simulink library "traj_lib"  (R2018b)
settings: Solver=VariableStepAuto  StartTime=0.0  StopTime=10.0  RelTol=1e-3
undefined symbols (not defined in the file or in its folder): traj_empty_struct, traj_params
libraries: $bdroot x1, simulink x1
settings Model: Creator=fabian  LastModifiedBy=yannic

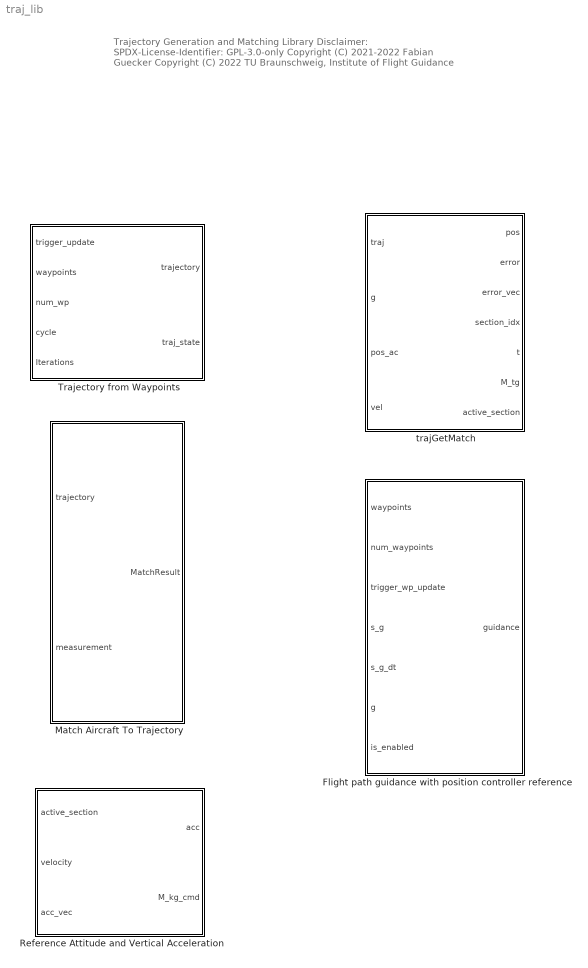
== system traj_lib ==
  note: Trajectory Generation and Matching Library
      |
      | Disclaimer:
      | SPDX-License-Identifier: GPL-3.0-only
      |
      | Copyright (C) 2021-2022 Fabian Guecker
      | Copyright (C) 2022 TU Braunschweig, Institute of Flight Guidance
  Flight path guidance with position controller reference : Subsystem  mask{traj_params=traj_params, T_inner_loop=0.1, mask_expr_handling_config=default}
      mask prompts: traj_params "Guided flight mode parameters struct"; T_inner_loop "Inner loop time constant seen by position controller, in s"
      mask init:
      | maskExprHandling(gcbh, mask_expr_handling_config);
      mask TypeOptions mask_expr_handling_config: default | passthrough (tunable)
      mask DialogControl DescGroupVar Prompt: Position controller reference from waypoints
      mask DialogControl DescTextVar Prompt: Waypoints are connected by splines. The shortest distance to the desired flight path is computed. Then the corresponding desired position, velocity and acceleration are computed based on the desired flight-path velocity.
      mask DialogControl CodeGenerationSettings Prompt: Code Generation Settings
      mask DialogControl maskExprHandlingText Prompt: Mask expression handling
      mask DialogControl maskExprHandlingReadme Prompt: README
      mask DialogControl maskExprHandlingReadme Tooltip: https://github.com/iff-gsc/m-Utils/tree/main/simulink/mask_expression_handling/README.md
      mask DialogControl maskExprHandlingReadme Callback: web('https://github.com/iff-gsc/m-Utils/tree/main/simulink/mask_expression_handling/README.md','-browser')
  Match Aircraft To Trajectory : Subsystem
      mask DialogControl DescGroupVar Prompt: Match Aircraft to Trajectory
  Reference Attitude and Vertical Acceleration : Subsystem  mask{G0=9.81}
      mask prompts: G0 "earth acceleration [m/s^2]"
  Trajectory from Waypoints : Subsystem  mask{traj_parameter=traj_params}
      mask prompts: traj_parameter "Trajectory parameters struct, see trajLoadParams"
      mask init:
      | [traj_empty_struct] = trajInit(traj_parameter.wpmax, traj_parameter.degree);
      | struct2slbus( traj_empty_struct, 'trajectoryStruct' );
      mask DialogControl DescGroupVar Prompt: Trajectory from Waypoints
  trajGetMatch : MATLAB Function  TreatAsAtomicUnit=on

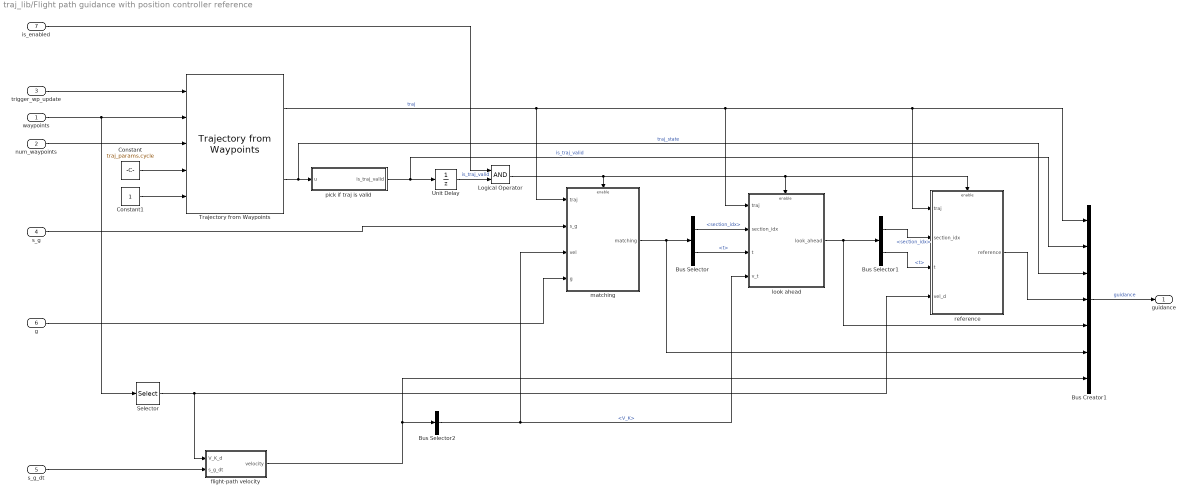
== system traj_lib/Flight path guidance with position controller reference ==
  waypoints : Inport
  num_waypoints : Inport  Port=2
  trigger_wp_update : Inport  Port=3
  s_g : Inport  Port=4
  s_g_dt : Inport  Port=5
  g : Inport  Port=6
  is_enabled : Inport  Port=7
  Bus Creator1 : BusCreator  Inputs=7
  Bus Selector : BusSelector  OutputSignals=section_idx,t
  Bus Selector1 : BusSelector  OutputSignals=section_idx,t
  Bus Selector2 : BusSelector  OutputSignals=V_K
  Constant : Constant  Value=traj_params.cycle
  Constant1 : Constant
  Logical Operator : Logic  AllPortsSameDT=off  OutDataTypeStr=boolean
  Selector : Selector  NumberOfDimensions=2  InputPortWidth=3  IndexOptions=Index vector (dialog),Index vector (dialog)  Indices=4,1  OutputSizes=1,1
  Trajectory from Waypoints : $bdroot/Trajectory from Waypoints  traj_parameter=traj_params
  Unit Delay : UnitDelay  SampleTime=-1
  flight-path velocity : Subsystem
  look ahead : Subsystem
  matching : Subsystem
  pick if traj is valid : MATLAB Function  TreatAsAtomicUnit=on
  reference : Subsystem
  guidance : Outport
  wires:
  waypoints/1 -> Selector/1, Trajectory from Waypoints/2
  g/1 -> matching/4(g)
  Constant/1 -> Trajectory from Waypoints/4
  Trajectory from Waypoints/1 -> matching/1(traj), look ahead/1(traj), reference/1(traj), Bus Creator1/1  "traj"
  s_g/1 -> matching/2(s_g)
  matching/1(matching) -> Bus Creator1/6, Bus Selector/1
  Selector/1 -> flight-path velocity/1(V_K_d), reference/4(vel_d)
  look ahead/1(look_ahead) -> Bus Creator1/5, Bus Selector1/1
  reference/1(reference) -> Bus Creator1/4
  Bus Selector/1 -> look ahead/2(section_idx)  "<section_idx>"
  Bus Selector/2 -> look ahead/3(t)  "<t>"
  Bus Selector1/1 -> reference/2(section_idx)  "<section_idx>"
  Bus Selector1/2 -> reference/3(t)  "<t>"
  Bus Creator1/1 -> guidance/1  "guidance"
  s_g_dt/1 -> flight-path velocity/2(s_g_dt)
  flight-path velocity/1(velocity) -> Bus Creator1/7, Bus Selector2/1
  Bus Selector2/1 -> look ahead/4(v_t), matching/3(vel)  "<V_K>"
  Constant1/1 -> Trajectory from Waypoints/5
  num_waypoints/1 -> Trajectory from Waypoints/3
  Trajectory from Waypoints/2 -> Bus Creator1/3, pick if traj is valid/1(u)  "traj_state"
  pick if traj is valid/1(is_traj_valid) -> Unit Delay/1, Bus Creator1/2  "is_traj_valid"
  Logical Operator/1 -> matching/Enable, look ahead/Enable, reference/Enable
  trigger_wp_update/1 -> Trajectory from Waypoints/1
  is_enabled/1 -> Logical Operator/1
  Unit Delay/1 -> Logical Operator/2  "is_traj_valid"

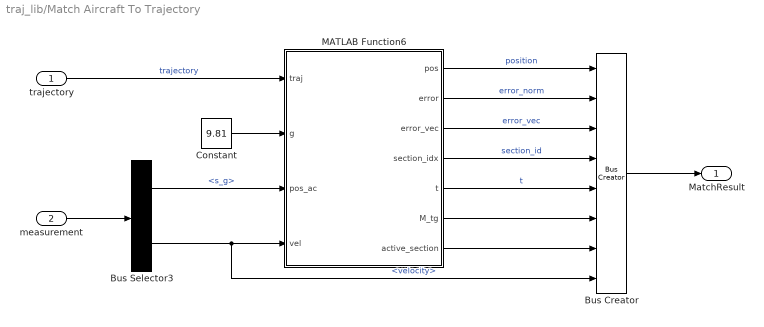
== system traj_lib/Match Aircraft To Trajectory ==
  trajectory : Inport
  measurement : Inport  Port=2
  Bus Creator : BusCreator  Inputs=8
  Bus Selector3 : BusSelector  OutputSignals=EKF.s_g,EKF.velocity
  Constant : Constant  Value=9.81
  MATLAB Function6 : MATLAB Function  TreatAsAtomicUnit=on
  MatchResult : Outport
  wires:
  Bus Selector3/1 -> MATLAB Function6/3(pos_ac)  "<s_g>"
  trajectory/1 -> MATLAB Function6/1(traj)  "trajectory"
  measurement/1 -> Bus Selector3/1
  Bus Creator/1 -> MatchResult/1
  Bus Selector3/2 -> Bus Creator/8, MATLAB Function6/4(vel)  "<velocity>"
  Constant/1 -> MATLAB Function6/2(g)
  MATLAB Function6/1(pos) -> Bus Creator/1  "position"
  MATLAB Function6/2(error) -> Bus Creator/2  "error_norm"
  MATLAB Function6/3(error_vec) -> Bus Creator/3  "error_vec"
  MATLAB Function6/4(section_idx) -> Bus Creator/4  "section_id"
  MATLAB Function6/5(t) -> Bus Creator/5  "t"
  MATLAB Function6/6(M_tg) -> Bus Creator/6
  MATLAB Function6/7(active_section) -> Bus Creator/7

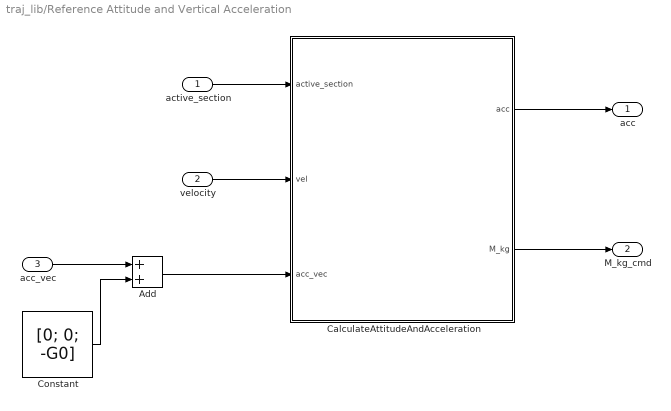
== system traj_lib/Reference Attitude and Vertical Acceleration ==
  active_section : Inport
  velocity : Inport  Port=2
  acc_vec : Inport  Port=3
  Add : Sum
  CalculateAttitudeAndAcceleration : MATLAB Function  TreatAsAtomicUnit=on
  Constant : Constant  Value=[0; 0; -G0]  VectorParams1D=off
  acc : Outport
  M_kg_cmd : Outport  Port=2
  wires:
  active_section/1 -> CalculateAttitudeAndAcceleration/1(active_section)
  velocity/1 -> CalculateAttitudeAndAcceleration/2(vel)
  CalculateAttitudeAndAcceleration/2(M_kg) -> M_kg_cmd/1
  Constant/1 -> Add/2
  CalculateAttitudeAndAcceleration/1(acc) -> acc/1
  acc_vec/1 -> Add/1
  Add/1 -> CalculateAttitudeAndAcceleration/3(acc_vec)

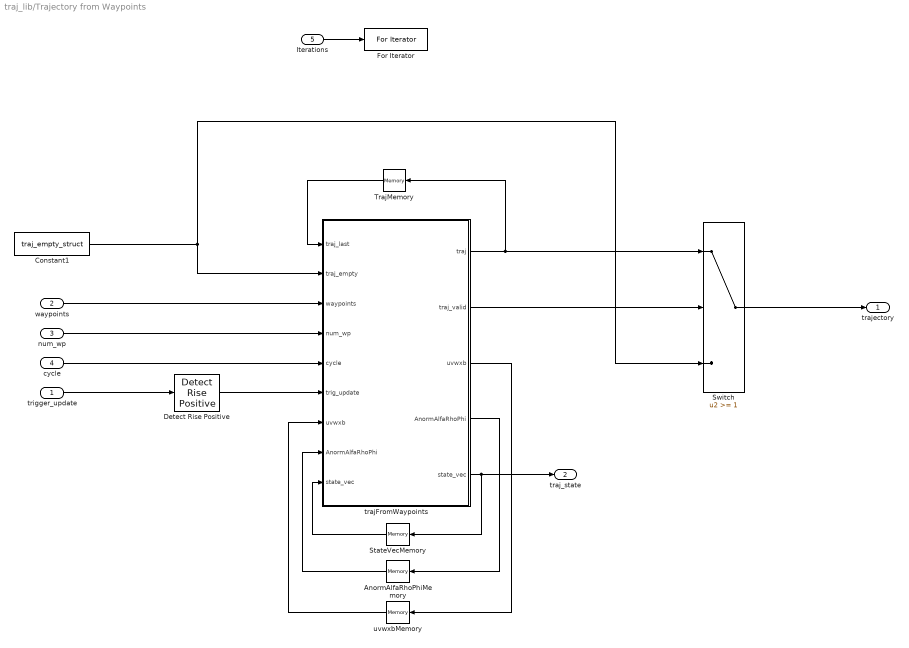
== system traj_lib/Trajectory from Waypoints ==
  trigger_update : Inport
  waypoints : Inport  Port=2
  num_wp : Inport  Port=3
  cycle : Inport  Port=4
  Iterations : Inport  Port=5  OutMin=[1]  OutMax=[100]  PortDimensions=1
  AnormAlfaRhoPhiMemory : Memory  InitialCondition=zeros(4,1)  InheritSampleTime=on
  Constant1 : Constant  Value=traj_empty_struct  OutDataTypeStr=Bus: trajectoryStructBus
  Detect Rise Positive : simulink/Logic and Bit Operations/Detect Rise Positive  vinit=0  OutDataTypeStr=boolean
  For Iterator : ForIterator  IterationSource=external  IterationLimit=100  ShowIterationPort=off
  "StateVecMemory " : Memory  InitialCondition=zeros(6,1)  InheritSampleTime=on
  Switch : Switch  Threshold=1
  TrajMemory : Memory  InitialCondition=traj_empty_struct  InheritSampleTime=on
  trajFromWaypoints : MATLAB Function  TreatAsAtomicUnit=on
  uvwxbMemory : Memory  InitialCondition=zeros(traj_parameter.wpmax*(traj_parameter.degree+1),5)  InheritSampleTime=on
  trajectory : Outport
  traj_state : Outport  Port=2
  wires:
  AnormAlfaRhoPhiMemory/1 -> trajFromWaypoints/8("AnormAlfaRhoPhi ")
  Switch/1 -> trajectory/1
  Iterations/1 -> For Iterator/1
  num_wp/1 -> trajFromWaypoints/4(num_wp)
  waypoints/1 -> trajFromWaypoints/3(waypoints)
  TrajMemory/1 -> trajFromWaypoints/1(traj_last)
  Detect Rise Positive/1 -> trajFromWaypoints/6(trig_update)
  cycle/1 -> trajFromWaypoints/5(cycle)
  Constant1/1 -> trajFromWaypoints/2(traj_empty), Switch/3
  uvwxbMemory/1 -> trajFromWaypoints/7("uvwxb ")
  "StateVecMemory "/1 -> trajFromWaypoints/9("state_vec ")
  trajFromWaypoints/5(state_vec) -> traj_state/1, "StateVecMemory "/1
  trajFromWaypoints/2(traj_valid) -> Switch/2
  trigger_update/1 -> Detect Rise Positive/1
  trajFromWaypoints/1(traj) -> TrajMemory/1, Switch/1
  trajFromWaypoints/4(AnormAlfaRhoPhi) -> AnormAlfaRhoPhiMemory/1
  trajFromWaypoints/3(uvwxb) -> uvwxbMemory/1

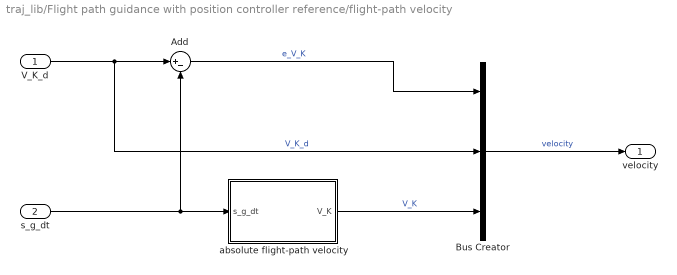
== system traj_lib/Flight path guidance with position controller reference/flight-path velocity ==
  V_K_d : Inport
  s_g_dt : Inport  Port=2
  Add : Sum  Inputs=|+-
  Bus Creator : BusCreator  Inputs=3
  absolute flight-path velocity : Subsystem
  velocity : Outport
  wires:
  s_g_dt/1 -> absolute flight-path velocity/1(s_g_dt), Add/2
  absolute flight-path velocity/1(V_K) -> Bus Creator/3  "V_K"
  V_K_d/1 -> Bus Creator/2, Add/1  "V_K_d"
  Bus Creator/1 -> velocity/1  "velocity"
  Add/1 -> Bus Creator/1  "e_V_K"

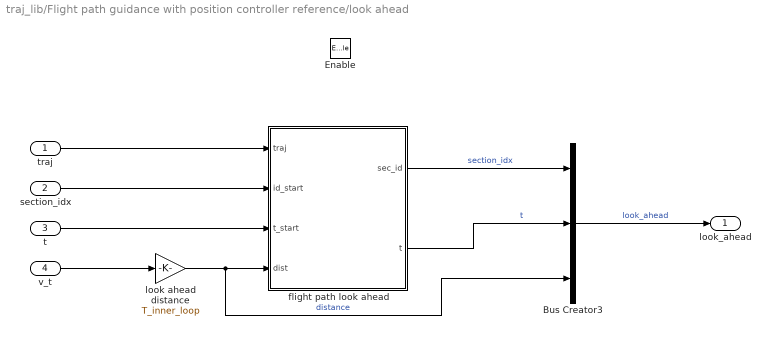
== system traj_lib/Flight path guidance with position controller reference/look ahead ==
  traj : Inport
  section_idx : Inport  Port=2
  t : Inport  Port=3
  v_t : Inport  Port=4
  Enable : EnablePort
  Bus Creator3 : BusCreator  Inputs=3
  flight path look ahead : MATLAB Function  TreatAsAtomicUnit=on
  look ahead distance : Gain  Gain=T_inner_loop
  look_ahead : Outport
  wires:
  v_t/1 -> look ahead distance/1
  flight path look ahead/2(t) -> Bus Creator3/2  "t"
  Bus Creator3/1 -> look_ahead/1  "look_ahead"
  section_idx/1 -> flight path look ahead/2(id_start)
  traj/1 -> flight path look ahead/1(traj)
  flight path look ahead/1(sec_id) -> Bus Creator3/1  "section_idx"
  t/1 -> flight path look ahead/3(t_start)
  look ahead distance/1 -> Bus Creator3/3, flight path look ahead/4(dist)  "distance"

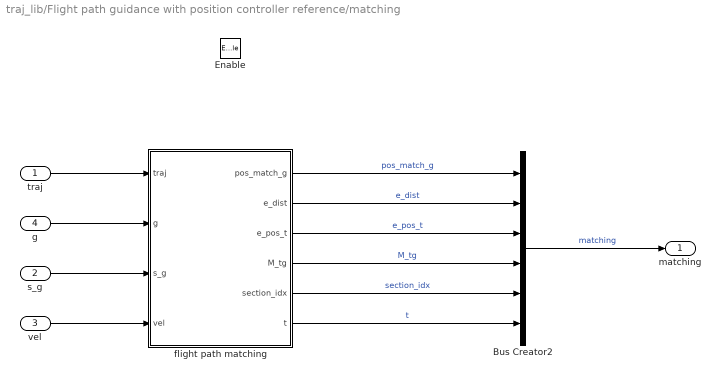
== system traj_lib/Flight path guidance with position controller reference/matching ==
  traj : Inport
  s_g : Inport  Port=2
  vel : Inport  Port=3
  g : Inport  Port=4
  Enable : EnablePort
  Bus Creator2 : BusCreator  Inputs=6
  flight path matching : MATLAB Function  TreatAsAtomicUnit=on
  matching : Outport
  wires:
  flight path matching/5(section_idx) -> Bus Creator2/5  "section_idx"
  traj/1 -> flight path matching/1(traj)
  flight path matching/3(e_pos_t) -> Bus Creator2/3  "e_pos_t"
  flight path matching/6(t) -> Bus Creator2/6  "t"
  g/1 -> flight path matching/2(g)
  flight path matching/1(pos_match_g) -> Bus Creator2/1  "pos_match_g"
  vel/1 -> flight path matching/4(vel)
  flight path matching/2(e_dist) -> Bus Creator2/2  "e_dist"
  s_g/1 -> flight path matching/3(s_g)
  Bus Creator2/1 -> matching/1  "matching"
  flight path matching/4(M_tg) -> Bus Creator2/4  "M_tg"

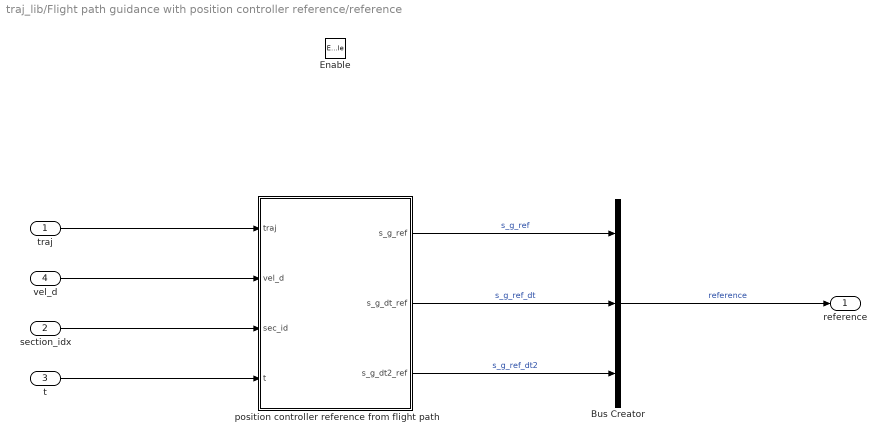
== system traj_lib/Flight path guidance with position controller reference/reference ==
  traj : Inport
  section_idx : Inport  Port=2
  t : Inport  Port=3
  vel_d : Inport  Port=4
  Enable : EnablePort
  Bus Creator : BusCreator  Inputs=3
  position controller reference from flight path : MATLAB Function  TreatAsAtomicUnit=on
  reference : Outport
  wires:
  position controller reference from flight path/1(s_g_ref) -> Bus Creator/1  "s_g_ref"
  vel_d/1 -> position controller reference from flight path/2(vel_d)
  position controller reference from flight path/2(s_g_dt_ref) -> Bus Creator/2  "s_g_ref_dt"
  t/1 -> position controller reference from flight path/4(t)
  position controller reference from flight path/3(s_g_dt2_ref) -> Bus Creator/3  "s_g_ref_dt2"
  traj/1 -> position controller reference from flight path/1(traj)
  Bus Creator/1 -> reference/1  "reference"
  section_idx/1 -> position controller reference from flight path/3(sec_id)

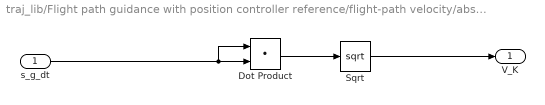
== system traj_lib/Flight path guidance with position controller reference/flight-path velocity/absolute flight-path velocity ==
  s_g_dt : Inport
  Dot Product : DotProduct  InputSameDT=on  OutDataTypeStr=Inherit: Inherit via internal rule
  Sqrt : Sqrt  SaturateOnIntegerOverflow=on
  V_K : Outport
  wires:
  Dot Product/1 -> Sqrt/1
  Sqrt/1 -> V_K/1
  s_g_dt/1 -> Dot Product/1, Dot Product/2

== matlab function traj_lib/trajGetMatch ==
  data: pos output; error output; error_vec output; traj input; g input; pos_ac input; section_idx output; t output; M_tg output; vel input; active_section output Bus: sections
function [pos, error, error_vec, section_idx, t, M_tg, active_section]  = GetMatch(traj, g, pos_ac, vel)

    section_idx = ones(1,superiorfloat(pos_ac));

    [section_idx, error, t] = trajGetMatchEnhanced(traj, pos_ac, section_idx);
    
    active_section   = trajGetSection(traj, section_idx);
    active_section.t = t;
    
    pos = trajSectionGetPos(active_section);
         
    error_vec = (pos - pos_ac);  

    [T, B, N, ~, ~] = trajSectionGetFrenetSerretWithGravity(active_section, vel, g);

    M_tg = [T, B, -N];

end

== matlab function traj_lib/Match Aircraft To Trajectory/MATLAB Function6 ==
  data: pos output; error output; error_vec output; traj input; g input; pos_ac input; section_idx output; t output; M_tg output; vel input; active_section output Bus: sections
function [pos, error, error_vec, section_idx, t, M_tg, active_section]  = GetMatch(traj, g, pos_ac, vel)

    section_idx = 1;

    [section_idx, error, t] = trajGetMatch(traj, pos_ac, section_idx);
    
    active_section   = trajGetSection(traj, section_idx);
    active_section.t = t;
    
    pos = trajSectionGetPos(active_section);
         
    error_vec = (pos - pos_ac);  

    [T, B, N, ~, ~] = trajSectionGetFrenetSerretWithGravity(active_section, vel, g);

    M_tg = [T, B, -N];

end

== matlab function traj_lib/Flight path guidance with position controller reference/pick if traj is valid ==
  data: u input; is_traj_valid output
function is_traj_valid = fcn(u)
is_traj_valid = u(5);
end

== matlab function traj_lib/Flight path guidance with position controller reference/matching/flight path matching ==
  data: pos_match_g output; e_dist output; e_pos_t output; M_tg output; traj input size=1; section_idx output size=1; g input size=1; s_g input size=3; vel input size=1; t output size=1
function [pos_match_g, e_dist, e_pos_t, M_tg, section_idx, t]  = fcn(traj, g, s_g, vel)

    [section_idx, e_dist, t] = trajGetMatchEnhanced(traj, s_g);
    
    traj_section   = trajGetSection(traj, section_idx);
    
    pos_match_g = trajSectionGetPos(traj_section,t);
    
    [T, B, N, ~, ~] = trajSectionGetFrenetSerretWithGravity(traj_section, vel, g, t);
    M_tg = [T, B, -N]';
         
    e_pos_t = M_tg * (pos_match_g - s_g);  
    
end

== matlab function traj_lib/Flight path guidance with position controller reference/reference/position controller reference from flight path ==
  data: traj input; vel_d input; s_g_ref output size=3; s_g_dt_ref output; sec_id input; t input; s_g_dt2_ref output
function [s_g_ref,s_g_dt_ref,s_g_dt2_ref] = fcn(traj, vel_d, sec_id, t)
traj_section = trajGetSection(traj,sec_id);
s_g_ref = trajSectionGetPos(traj_section,t);
s_g_dt_ref = trajSectionGetVel(traj_section,vel_d,t);
s_g_dt2_ref = trajSectionGetAcc(traj_section,vel_d,0, t);
end

== matlab function traj_lib/Flight path guidance with position controller reference/look ahead/flight path look ahead ==
  data: traj input; sec_id output size=1; id_start input size=1; t_start input; dist input; t output size=1
function [sec_id,t] = trajSweepAlong(traj,id_start,t_start,dist)
[sec_id, t] = trajSweepAlong(traj,id_start,t_start,dist);
end

== matlab function traj_lib/Reference Attitude and Vertical Acceleration/CalculateAttitudeAndAcceleration ==
  data: active_section input; vel input; acc output; M_kg output; acc_vec input
function [acc, M_kg] = CalculateAttitudeAndAcceleration(active_section, vel, acc_vec)

[T, B, N, kappa, ~] = trajSectionGetFrenetSerretWithAcceleration(active_section, vel, acc_vec);

% Calculate path acceleration
acc = (kappa * N) * vel^2;

M_kg = [T, B, -N];

end

== matlab function traj_lib/Trajectory from Waypoints/trajFromWaypoints ==
  settings: updateMethod=DISCRETE
  data: traj_last input; traj_empty input; waypoints input; num_wp input; cycle input; trig_update input; uvwxb input; AnormAlfaRhoPhi input; traj output Bus: trajectoryStructBus; traj_valid output; uvwxb output; AnormAlfaRhoPhi output; state_vec input; state_vec output; traj_empty_struct parameter
function [traj, traj_valid, uvwxb, AnormAlfaRhoPhi, state_vec] = ...
    trajFromWaypointsIterative(traj_last,traj_empty,waypoints,num_wp, ...
    cycle,trig_update,uvwxb,AnormAlfaRhoPhi,state_vec,traj_empty_struct)

[traj, traj_valid, uvwxb, AnormAlfaRhoPhi, state_vec] = ...
    trajFromWaypointsIterative(traj_last,traj_empty,waypoints,num_wp, ...
    cycle,trig_update,uvwxb,AnormAlfaRhoPhi,state_vec,traj_empty_struct);

end
